simulink model "B7_Driver"  (R2022b)
settings: Solver=FixedStepDiscrete  StartTime=0.0  StopTime=10  FixedStep=Ts  RelTol=1e-3
values from neighbouring files (symbols this model uses):
  Ts = 0.01    [build_B2_AutoHeadlamp.m]    (also in build_B3_AHB.m)
undefined symbols (not defined in the file or in its folder): POS_DIM, T_SOFT, TAIL_DIM, V_EFF
settings Model: Creator=LENOVO  LastModifiedBy=LENOVO

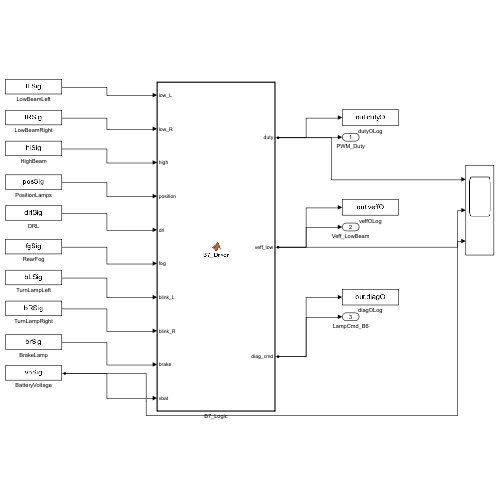
[thumbnail: Simulink's stored preview of the top-level diagram]
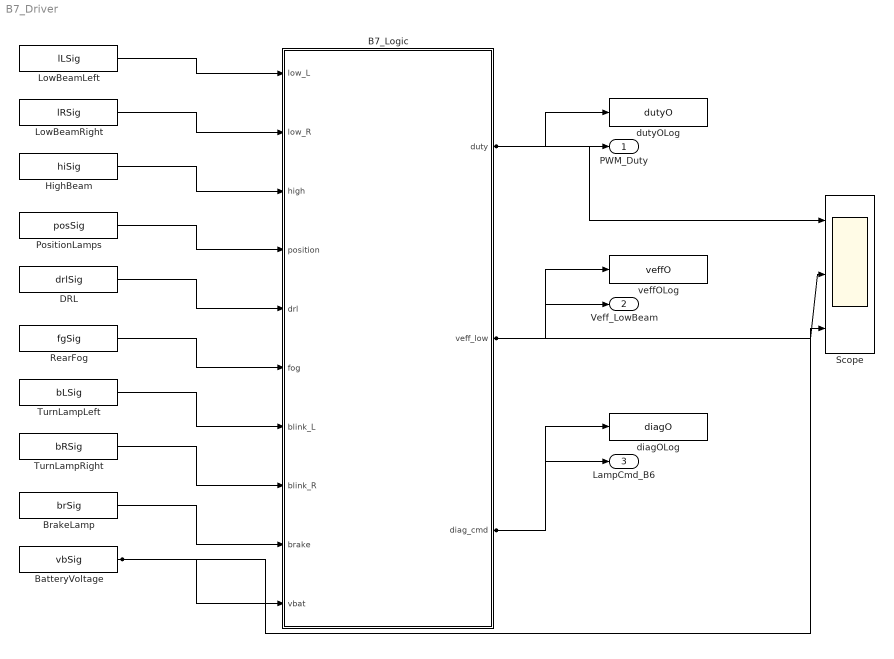
== system B7_Driver ==
  B7_Logic : MATLAB Function  TreatAsAtomicUnit=on
  BatteryVoltage : FromWorkspace  VariableName=vbSig  SampleTime=Ts  OutputAfterFinalValue=Holding final value
  BrakeLamp : FromWorkspace  VariableName=brSig  SampleTime=Ts  Interpolate=off  OutputAfterFinalValue=Holding final value
  DRL : FromWorkspace  VariableName=drlSig  SampleTime=Ts  Interpolate=off  OutputAfterFinalValue=Holding final value
  HighBeam : FromWorkspace  VariableName=hiSig  SampleTime=Ts  Interpolate=off  OutputAfterFinalValue=Holding final value
  LowBeamLeft : FromWorkspace  VariableName=lLSig  SampleTime=Ts  Interpolate=off  OutputAfterFinalValue=Holding final value
  LowBeamRight : FromWorkspace  VariableName=lRSig  SampleTime=Ts  Interpolate=off  OutputAfterFinalValue=Holding final value
  PositionLamps : FromWorkspace  VariableName=posSig  SampleTime=Ts  Interpolate=off  OutputAfterFinalValue=Holding final value
  RearFog : FromWorkspace  VariableName=fgSig  SampleTime=Ts  Interpolate=off  OutputAfterFinalValue=Holding final value
  Scope : Scope  NumInputPorts=3
  TurnLampLeft : FromWorkspace  VariableName=bLSig  SampleTime=Ts  Interpolate=off  OutputAfterFinalValue=Holding final value
  TurnLampRight : FromWorkspace  VariableName=bRSig  SampleTime=Ts  Interpolate=off  OutputAfterFinalValue=Holding final value
  diagOLog : ToWorkspace  VariableName=diagO  SaveFormat=Timeseries  SampleTime=-1
  dutyOLog : ToWorkspace  VariableName=dutyO  SaveFormat=Timeseries  SampleTime=-1
  veffOLog : ToWorkspace  VariableName=veffO  SaveFormat=Timeseries  SampleTime=-1
  PWM_Duty : Outport
  Veff_LowBeam : Outport  Port=2
  LampCmd_B6 : Outport  Port=3
  wires:
  LowBeamLeft/1 -> B7_Logic/1(low_L)
  LowBeamRight/1 -> B7_Logic/2(low_R)
  HighBeam/1 -> B7_Logic/3(high)
  PositionLamps/1 -> B7_Logic/4(position)
  DRL/1 -> B7_Logic/5(drl)
  RearFog/1 -> B7_Logic/6(fog)
  TurnLampLeft/1 -> B7_Logic/7(blink_L)
  TurnLampRight/1 -> B7_Logic/8(blink_R)
  BrakeLamp/1 -> B7_Logic/9(brake)
  BatteryVoltage/1 -> B7_Logic/10(vbat), Scope/3
  B7_Logic/1(duty) -> dutyOLog/1, PWM_Duty/1, Scope/1
  B7_Logic/2(veff_low) -> veffOLog/1, Veff_LowBeam/1, Scope/2
  B7_Logic/3(diag_cmd) -> diagOLog/1, LampCmd_B6/1

== matlab function B7_Driver/B7_Logic ==
  data: low_L input; duty output; low_R input; high input; position input; drl input; fog input; blink_L input; blink_R input; brake input; vbat input; veff_low output; diag_cmd output; Ts parameter; V_EFF parameter; T_SOFT parameter; POS_DIM parameter; TAIL_DIM parameter
function [duty, veff_low, diag_cmd] = B7_Driver(low_L, low_R, high, position, drl, fog, blink_L, blink_R, brake, vbat, Ts, V_EFF, T_SOFT, POS_DIM, TAIL_DIM)
%#codegen
% B7 - Pilotage des sorties (PWM)
% duty (8 voies, %) : 1 croisement G, 2 croisement D, 3 route, 4 LED avant DRL/veilleuse,
%                     5 clignotant G, 6 clignotant D, 7 LED arriere stop/position, 8 antibrouillard AR
persistent ramp
if isempty(ramp), ramp = zeros(4,1); end         % rampes : croisement G, croisement D, route, antibrouillard

% 1) Regulation de tension des lampes halogenes : tension efficace constante = V_EFF
d_reg = min(1, (V_EFF / max(vbat, 1))^2);         % Veff = sqrt(duty) * Vbat

% 2) Demarrage progressif (soft-start) : limite le pic de courant du filament froid
req = [low_L; low_R; high; fog];
for i = 1:4
    if req(i)
        ramp(i) = min(ramp(i) + Ts / T_SOFT, 1);  % 0 -> 100 % en T_SOFT
    else
        ramp(i) = 0;                              % extinction immediate
    end
end
d = zeros(8,1);
d(1) = ramp(1) * d_reg;  d(2) = ramp(2) * d_reg;  d(3) = ramp(3) * d_reg;  d(8) = ramp(4) * d_reg;

% 3) LED avant a deux niveaux : DRL plein (100 %), veilleuse attenuee (REQ-LSC-05)
if drl
    d(4) = 1;
elseif position
    d(4) = POS_DIM;
end
% 4) Clignotants : pleine tension regulee des le 1er pas (pas de rampe, flash net)
d(5) = double(blink_L) * d_reg;  d(6) = double(blink_R) * d_reg;
% 5) LED arriere a deux niveaux : stop plein, position attenuee
if brake
    d(7) = 1;
elseif position
    d(7) = TAIL_DIM;
end

duty     = uint8(round(100 * d));
veff_low = sqrt(d(1)) * vbat;                     % tension efficace vue par le croisement gauche
diag_cmd = [d(1) > 0; d(2) > 0; d(5) > 0; d(6) > 0];   % lampes allumees, pour le diagnostic B6
